simulink model "DiSiUp_1lab_3"  (R2025b)
settings: Solver=VariableStepAuto  StartTime=0.0  StopTime=100  RelTol=1e-8
values from neighbouring files (symbols this model uses):
  B_gen = [0; 0]    [DiSiUp_1lab_3_mat.m]
  D_gen = 0    [DiSiUp_1lab_3_mat.m]
  Gamma_d = [cos(T*omega),  sin(T*omega) ... (first row only)    [DiSiUp_1lab_3_mat.m]
  H = [A_sig, 0]    [DiSiUp_1lab_3_mat.m]
  T = 0.2    [DiSiUp_1lab_3_mat.m]
  xi0 = [0; 1]    [DiSiUp_1lab_3_mat.m]
settings Model: Creator=waltanmari  LastModifiedBy=waltanmari

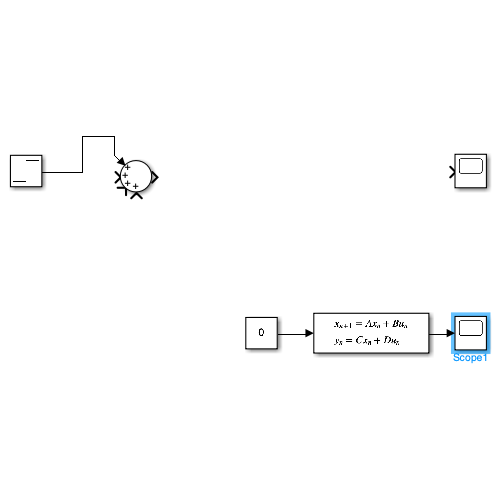
[thumbnail: Simulink's stored preview of the top-level diagram]
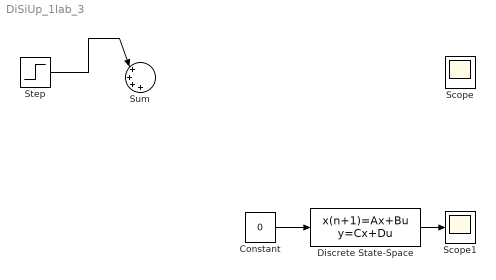
== system DiSiUp_1lab_3 ==
  Constant : Constant  Value=0
  Discrete State-Space : DiscreteStateSpace  A=Gamma_d  B=B_gen  C=H  D=D_gen  InitialCondition=xi0  SampleTime=T
  Scope : Scope
      settings: ActiveDisplayYMinimum=-1  ActiveDisplayYMaximum=1
  Scope1 : Scope
      settings: ActiveDisplayYMinimum=-0.606776920085166  ActiveDisplayYMaximum=0.067419657787240655
  Step : Step  Time=0  After=0  SampleTime=0
  Sum : Sum  Inputs=|++++
  wires:
  Step/1 -> Sum/1
  Constant/1 -> Discrete State-Space/1
  Discrete State-Space/1 -> Scope1/1
